simulink subsystem "Electromechanical"  (R2025b)
settings: Solver=VariableStepAuto
undefined symbols (not defined in the file): motor
settings Model: Creator=Compu  LastModifiedBy=ahmed medhat

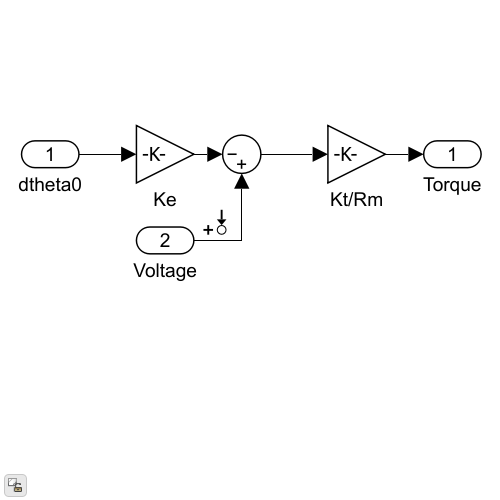
[thumbnail: Simulink's stored preview of the top-level diagram]
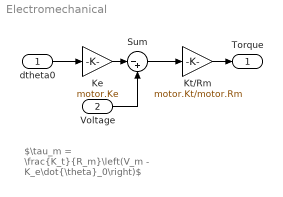
== system Electromechanical ==
  note: $\tau_m = \frac{K_t}{R_m}\left(V_m - K_e\dot{\theta}_0\right)$
  dtheta0 : Inport
  Voltage : Inport  Port=2
  Ke : Gain  Gain=motor.Ke
  Kt/Rm : Gain  Gain=motor.Kt/motor.Rm
  Sum : Sum  Inputs=|-+
  Torque : Outport
  wires:
  Voltage/1 -> Sum/2
  dtheta0/1 -> Ke/1
  Ke/1 -> Sum/1
  Sum/1 -> Kt/Rm/1
  Kt/Rm/1 -> Torque/1
